simulink model "MMC_phase_centralized_HAAS_20260927"  (R2024b)
settings: Solver=FixedStepDiscrete  StartTime=t_init_sim  StopTime=sim_time  FixedStep=Ts  RelTol=1e-3
values from neighbouring files (symbols this model uses):
  a = 1    [script_MMC_phase_hackathon_NLM_centralized_HAAS_20260927.m]
  C1low1_active = 1    [script_MMC_phase_hackathon_NLM_centralized_HAAS_20260927.m]
  C2low1_active = 1    [script_MMC_phase_hackathon_NLM_centralized_HAAS_20260927.m]
  C_bus = 4400e-6    (= 0.0044)    [script_MMC_phase_hackathon_NLM_centralized_HAAS_20260927.m]
  C_M_extra = C_m-twist_high_side_C    [script_MMC_phase_hackathon_NLM_centralized_HAAS_20260927.m]
  duty_cycle = 1.0    (= 1)    [script_MMC_phase_hackathon_NLM_centralized_HAAS_20260927.m]
  f0 = 50    [script_MMC_phase_hackathon_NLM_centralized_HAAS_20260927.m]
  feeder_current_lower_rate_limit = -10    [script_MMC_phase_hackathon_NLM_centralized_HAAS_20260927.m]    (also in twist_parameters.m = -500)
  feeder_current_tab = [0.328 0.217 0.162 0.132 0.109 0.094 0.083 0.075 0.068 0.062 0.058 0.054 ... (42 elements, 14x3)]    [feeder_current.mat]
  feeder_current_upper_rate_limit = 0.386/(20e-3)    (= 19.3)    [twist_parameters.m]
  is6VExternallySupplied = true    [script_MMC_phase_hackathon_NLM_centralized_HAAS_20260927.m]
  isFeederJumperOpen = true    [script_MMC_phase_hackathon_NLM_centralized_HAAS_20260927.m]
  L_arm = 30e-3    (= 0.03)    [script_MMC_phase_hackathon_NLM_centralized_HAAS_20260927.m]
  m = 1    [script_MMC_phase_hackathon_NLM_centralized_HAAS_20260927.m]
  N = 5    [script_MMC_phase_hackathon_NLM_centralized_HAAS_20260927.m]
  power_losses = false    [script_MMC_phase_hackathon_NLM_centralized_HAAS_20260927.m]
  R = 15    [script_MMC_phase_hackathon_NLM_centralized_HAAS_20260927.m]
  R_arm = 0.2    [script_MMC_phase_hackathon_NLM_centralized_HAAS_20260927.m]
  source_V = 0    [script_MMC_phase_hackathon_NLM_centralized_HAAS_20260927.m]
  Tcom_sample = round(Tcom / Ts)    [script_MMC_phase_hackathon_NLM_centralized_HAAS_20260927.m]
  time_charge = 0.1    [script_MMC_phase_hackathon_NLM_centralized_HAAS_20260927.m]
  time_decharge = 1.5    [script_MMC_phase_hackathon_NLM_centralized_HAAS_20260927.m]
  Ts = 1e-6    (= 1e-06)    [script_MMC_phase_hackathon_NLM_centralized_HAAS_20260927.m]
  twist_data_acquisition_delay = 50e-9    (= 5e-08)    [script_MMC_phase_hackathon_NLM_centralized_HAAS_20260927.m]    (also in twist_parameters.m)
  twist_data_sampling_period = 1/twist_freq_data_sampling    (= 5e-05)    [script_MMC_phase_hackathon_NLM_centralized_HAAS_20260927.m]    (also in twist_parameters.m)
  twist_dead_time = 200e-9    (= 2e-07)    [twist_parameters.m]
  twist_freq_switching = 200e3    (= 200000)    [twist_parameters.m]
  twist_high_side_adc_R = 1/(1/2e6 + 1/2e6 + 1/(330e3+5.6e3))    (= 251272.836178)    [twist_parameters.m]
  twist_high_side_C = 33e-6*4 + 4.7e-6*12    (= 0.0001884)    [twist_parameters.m]
  twist_high_side_feeder_R = 47e3+4.7e3    (= 51700)    [twist_parameters.m]
  twist_high_side_rC = 0.1    [twist_parameters.m]
  twist_low_side_adc_R = 150e3+470    (= 150470)    [twist_parameters.m]
  twist_low_side_C_ceramic = 3*4.7e-6    (= 1.41e-05)    [twist_parameters.m]
  twist_low_side_C_electrolytic = 47e-6    (= 4.7e-05)    [twist_parameters.m]
  twist_low_side_L = 33e-6    (= 3.3e-05)    [twist_parameters.m]
  twist_low_side_rC = 700e-3    (= 0.7)    [twist_parameters.m]
  twist_low_side_rL = 20e-3    (= 0.02)    [twist_parameters.m]
  twist_R_VCC = (tau_VCC/twist_high_side_C  - twist_high_side_rC)/(1-(tau_VCC/twist_high_side_C - twist_high_side_rC)/R_parallel)    (= 1110.74997822)    [twist_parameters.m]
  VDC = 48    [script_MMC_phase_hackathon_NLM_centralized_HAAS_20260927.m]
undefined symbols (not defined in the file or in its folder): C_SM, feeder_current, gcbh, sps_rtmsupport, twist_low_side_lC
libraries: spsSeriesRLCBranchLib x135, spsTriangleGeneratorLib x60, spsMosfetLib x60, spsCurrentMeasurementLib x43, spsVoltageMeasurementLib x35, spsControlledCurrentSourceLib x30, spsDiodeLib x22, spsIdealSwitchLib x20, spsControlledVoltageSourceLib x1, spsGroundLib x1, spspowerguiLib x1
(part 22 of 22)

== matlab function MMC_phase_centralized_HAAS_20260927/ /Communication_subsystem/Upper_arm/M1_Comm/Snapshot ==
  data: rx_signal input uint64; local_frame_snapshot input; rx_variables output single; sync input; round_done input
function rx_variables = Snapshot_block(rx_signal, local_frame_snapshot, sync, round_done)
%#codegen
%
% Snapshot block SSAF.
%
% Comportement voulu :
%   - pendant le round, les trames reçues mettent à jour working_bank ;
%   - local_frame_snapshot met à jour la donnée locale ;
%   - au front montant de sync, published_snapshot = working_bank ;
%   - le contrôle lit published_snapshot pendant la période de contrôle.
%
% round_done est conservé dans l'interface pour debug, mais la publication
% du snapshot se fait sur le front montant de sync.

% =========================
% Paramètres
% =========================
VC_LSB = single(0.1);
I_LSB  = single(0.1);

% =========================
% Etats persistants
% =========================
persistent working_bank
persistent published_snapshot
persistent sync_z
persistent last_rx_word
persistent last_rx_valid

if isempty(working_bank)
    working_bank = zeros(12, 1, 'single');
end

if isempty(published_snapshot)
    published_snapshot = zeros(12, 1, 'single');
end

if isempty(sync_z)
    sync_z = false;
end

if isempty(last_rx_word)
    last_rx_word = uint64(0);
end

if isempty(last_rx_valid)
    last_rx_valid = false;
end

% =========================
% Détection fronts sync
% =========================
sync_bool = sync ~= 0;
rise_sync = sync_bool && ~sync_z;

% =========================================================
% 1) Publication du snapshot au front montant
%
% Important :
%   published_snapshot est mis à jour AVANT la sortie.
%   Il contient les données reçues jusqu'au pas précédent.
%   Une trame qui arrive exactement au même pas que rise_sync est traitée
%   plus bas et sera donc visible au prochain front montant.
% =========================================================
if rise_sync
    published_snapshot = working_bank;
end

% =========================================================
% 2) Sortie enregistrée
%
% rx_variables ne dépend pas directement de rx_signal ou
% local_frame_snapshot au même pas de simulation.
% Cela évite une boucle algébrique avec le CVB.
% =========================================================
rx_variables = published_snapshot;

% Petit usage de round_done pour éviter qu'il soit complètement inutilisé.
% Il ne déclenche pas la publication.
if round_done ~= 0
    published_snapshot = published_snapshot;
end

% =========================
% 3) Mise à jour avec la trame locale
%
% local_frame_snapshot est émis seulement quand un nouveau round démarre.
% =========================
local_word = uint64(local_frame_snapshot(1));

[local_valid, local_current_present, local_id, local_vc, local_iarm] = ...
    unpack_frame(local_word, VC_LSB, I_LSB);

if local_valid
    working_bank = update_bank_from_frame(working_bank, ...
                                          local_valid, ...
                                          local_current_present, ...
                                          local_id, ...
                                          local_vc, ...
                                          local_iarm);
end

% =========================
% 4) Mise à jour avec la trame reçue depuis l'anneau
% =========================
rx_word = uint64(rx_signal(1));

[rx_valid, rx_current_present, rx_id, rx_vc, rx_iarm] = ...
    unpack_frame(rx_word, VC_LSB, I_LSB);

new_rx = rx_valid && ((rx_word ~= last_rx_word) || ~last_rx_valid);

if new_rx
    working_bank = update_bank_from_frame(working_bank, ...
                                          rx_valid, ...
                                          rx_current_present, ...
                                          rx_id, ...
                                          rx_vc, ...
                                          rx_iarm);
end

% =========================
% Mise à jour mémoires
% =========================
sync_z = sync_bool;

last_rx_word  = rx_word;
last_rx_valid = rx_valid;


% =========================================================
% UPDATE BANK FROM FRAME
% =========================================================
function bank_out = update_bank_from_frame(bank_in, valid, current_present, id, vc, iarm)
%#codegen

    bank_out = bank_in;

    if ~valid
        return;
    end

    % Upper arm : ID 1 à 5
    if id >= uint8(1) && id <= uint8(5)

        idx = double(id);          % ID 1 -> bank(1), ..., ID 5 -> bank(5)
        bank_out(idx) = single(vc);

        % Seul M1 transporte I_u
        if id == uint8(1) && current_present
            bank_out(6) = single(iarm);
        end

    % Lower arm : ID 6 à 10
    elseif id >= uint8(6) && id <= uint8(10)

        idx = 6 + double(id - uint8(5));  % ID 6 -> bank(7), ..., ID 10 -> bank(11)
        bank_out(idx) = single(vc);

        % Seul M6 transporte I_l
        if id == uint8(6) && current_present
            bank_out(12) = single(iarm);
        end
    end
end


% =========================================================
% UNPACK FRAME
%
% Format uint64:
%   bit 41      : valid
%   bit 40      : current_present
%   bits 39..32 : node_id
%   bits 31..16 : Vc local, uint16
%   bits 15..0  : I arm, int16 encodé en complément à deux
% =========================================================
function [valid, current_present, id, vc, iarm] = unpack_frame(frame, vc_lsb, i_lsb)
%#codegen

    frame_scalar = uint64(frame(1));

    valid = bitand(bitshift(frame_scalar, -41), uint64(1)) ~= uint64(0);
    current_present = bitand(bitshift(frame_scalar, -40), uint64(1)) ~= uint64(0);

    id = uint8(bitand(bitshift(frame_scalar, -32), uint64(255)));

    vc_q = uint16(bitand(bitshift(frame_scalar, -16), uint64(65535)));
    vc = single(double(vc_q) * double(vc_lsb));

    i_u16 = uint16(bitand(frame_scalar, uint64(65535)));

    if i_u16 >= uint16(32768)
        i_q_double = double(i_u16) - 65536;
    else
        i_q_double = double(i_u16);
    end

    iarm = single(i_q_double * double(i_lsb));
end

end

== matlab function MMC_phase_centralized_HAAS_20260927/ /Subsystem/Subsystem1/Hardware M4/Power losses branch 1/Branch switching loss ==
  data: VHigh input; twist_FET_Psw output; ILow input
function twist_FET_Psw = powerLossesSwitch(VHigh, ILow)
    %Twist switch power losses
    twist_freq_switching = 200e3;
    twist_FET_trise = 17e-9;
    twist_FET_tfall = 9e-9;

    twist_FET_Psw = 1/2*VHigh*ILow*twist_freq_switching*(twist_FET_trise + twist_FET_tfall);
end

== matlab function MMC_phase_centralized_HAAS_20260927/ /Subsystem/Subsystem1/Hardware M4/Power losses branch 2/Branch DT loss ==
  data: twist_FET_Pdt output; ILow input
function twist_FET_Pdt = powerLossesDeadTime(ILow)
    %Twist gate power losses
    twist_freq_switching = 200e3;
    twist_FET_Vf = 1.2;
    twist_FET_tDr = 10e-9;
    twist_FET_tDf = 0;

    twist_FET_Pdt = twist_FET_Vf*ILow*(twist_FET_tDr+twist_FET_tDf)*twist_freq_switching;
end

== matlab function MMC_phase_centralized_HAAS_20260927/ /Subsystem/Subsystem/Hardware M2/Feeder block/MATLAB Function ==
  data: i_feeder input; vC input; isfeederdisabled input; active_1 input; y output; Q_VCC output
function [y,Q_VCC]  = feeder_characteristics(i_feeder,vC,isfeederdisabled,active_1)

if(isfeederdisabled == 1)
    if(vC>=9.7)
        y = 11.2e-3;
        Q_VCC = 0;
    elseif(vC>=8.9 && vC < 9.7)
        if(active_1 == true)
            y = 11.2e-3;
            Q_VCC = 0;
        else
            y = 0;
            Q_VCC = 1;
        end
    else
        y = 0;
        Q_VCC = 1;
    end
else
    if(vC>=9.7)
        y = i_feeder;
        Q_VCC = 0;
    elseif(vC>=8.9 && vC < 9.7)
        if(active_1 == true)
            y = i_feeder;
            Q_VCC = 0;
        else
            y = 0;
            Q_VCC = 1;
        end
    else
        y = 0;
        Q_VCC = 1;
    end
end

== matlab function MMC_phase_centralized_HAAS_20260927/ /Subsystem/Subsystem1/Hardware M4/Power losses branch 2/Branch cond loss ==
  data: twist_FET_Pcond output; VHigh input; VLow input; ILow input
function twist_FET_Pcond = powerLossesCond(VHigh, VLow, ILow)
    %Twist conduction power losses
    twist_FET_Ron = 0.025;

    twist_FET_PcondH = pow2(ILow)*twist_FET_Ron*(VLow/VHigh);
    twist_FET_PcondL = pow2(ILow)*twist_FET_Ron*(1 - VLow/VHigh);

    twist_FET_Pcond = twist_FET_PcondH + twist_FET_PcondL;
end

== matlab function MMC_phase_centralized_HAAS_20260927/ /Subsystem/Subsystem1/Hardware M4/Power losses branch 2/Branch gate loss ==
  data: twist_FET_Pg output
function twist_FET_Pg = powerLossesGate()
    %Twist gate power losses
    twist_freq_switching = 200e3;
    twist_FET_QgH = 31e-9;
    twist_FET_QgL = 31e-9;
    twist_FET_Vgs = 11;

    twist_FET_Pg = (twist_FET_QgH + twist_FET_QgL)*twist_FET_Vgs*twist_freq_switching;
end

== matlab function MMC_phase_centralized_HAAS_20260927/ /Subsystem/Subsystem1/Hardware M4/Power losses branch 2/Branch switching loss ==
  data: VHigh input; twist_FET_Psw output; ILow input
function twist_FET_Psw = powerLossesSwitch(VHigh, ILow)
    %Twist switch power losses
    twist_freq_switching = 200e3;
    twist_FET_trise = 17e-9;
    twist_FET_tfall = 9e-9;

    twist_FET_Psw = 1/2*VHigh*ILow*twist_freq_switching*(twist_FET_trise + twist_FET_tfall);
end

== matlab function MMC_phase_centralized_HAAS_20260927/ /Subsystem/Subsystem1/Hardware M5/Feeder block/MATLAB Function ==
  data: i_feeder input; vC input; isfeederdisabled input; active_1 input; y output; Q_VCC output
function [y,Q_VCC]  = feeder_characteristics(i_feeder,vC,isfeederdisabled,active_1)

if(isfeederdisabled == 1)
    if(vC>=9.7)
        y = 11.2e-3;
        Q_VCC = 0;
    elseif(vC>=8.9 && vC < 9.7)
        if(active_1 == true)
            y = 11.2e-3;
            Q_VCC = 0;
        else
            y = 0;
            Q_VCC = 1;
        end
    else
        y = 0;
        Q_VCC = 1;
    end
else
    if(vC>=9.7)
        y = i_feeder;
        Q_VCC = 0;
    elseif(vC>=8.9 && vC < 9.7)
        if(active_1 == true)
            y = i_feeder;
            Q_VCC = 0;
        else
            y = 0;
            Q_VCC = 1;
        end
    else
        y = 0;
        Q_VCC = 1;
    end
end

== matlab function MMC_phase_centralized_HAAS_20260927/ /Subsystem/Subsystem1/Hardware M5/Power losses branch 1/Branch DT loss ==
  data: twist_FET_Pdt output; ILow input
function twist_FET_Pdt = powerLossesDeadTime(ILow)
    %Twist gate power losses
    twist_freq_switching = 200e3;
    twist_FET_Vf = 1.2;
    twist_FET_tDr = 10e-9;
    twist_FET_tDf = 0;

    twist_FET_Pdt = twist_FET_Vf*ILow*(twist_FET_tDr+twist_FET_tDf)*twist_freq_switching;
end

== matlab function MMC_phase_centralized_HAAS_20260927/ /Subsystem/Subsystem1/Hardware M5/Power losses branch 1/Branch cond loss ==
  data: twist_FET_Pcond output; VHigh input; VLow input; ILow input
function twist_FET_Pcond = powerLossesCond(VHigh, VLow, ILow)
    %Twist conduction power losses
    twist_FET_Ron = 0.025;

    twist_FET_PcondH = pow2(ILow)*twist_FET_Ron*(VLow/VHigh);
    twist_FET_PcondL = pow2(ILow)*twist_FET_Ron*(1 - VLow/VHigh);

    twist_FET_Pcond = twist_FET_PcondH + twist_FET_PcondL;
end

== matlab function MMC_phase_centralized_HAAS_20260927/ /Subsystem/Subsystem1/Hardware M5/Power losses branch 1/Branch gate loss ==
  data: twist_FET_Pg output
function twist_FET_Pg = powerLossesGate()
    %Twist gate power losses
    twist_freq_switching = 200e3;
    twist_FET_QgH = 31e-9;
    twist_FET_QgL = 31e-9;
    twist_FET_Vgs = 11;

    twist_FET_Pg = (twist_FET_QgH + twist_FET_QgL)*twist_FET_Vgs*twist_freq_switching;
end

== matlab function MMC_phase_centralized_HAAS_20260927/ /Subsystem/Subsystem1/Hardware M5/Power losses branch 1/Branch switching loss ==
  data: VHigh input; twist_FET_Psw output; ILow input
function twist_FET_Psw = powerLossesSwitch(VHigh, ILow)
    %Twist switch power losses
    twist_freq_switching = 200e3;
    twist_FET_trise = 17e-9;
    twist_FET_tfall = 9e-9;

    twist_FET_Psw = 1/2*VHigh*ILow*twist_freq_switching*(twist_FET_trise + twist_FET_tfall);
end

== matlab function MMC_phase_centralized_HAAS_20260927/ /Subsystem/Subsystem1/Hardware M5/Power losses branch 2/Branch DT loss ==
  data: twist_FET_Pdt output; ILow input
function twist_FET_Pdt = powerLossesDeadTime(ILow)
    %Twist gate power losses
    twist_freq_switching = 200e3;
    twist_FET_Vf = 1.2;
    twist_FET_tDr = 10e-9;
    twist_FET_tDf = 0;

    twist_FET_Pdt = twist_FET_Vf*ILow*(twist_FET_tDr+twist_FET_tDf)*twist_freq_switching;
end

== matlab function MMC_phase_centralized_HAAS_20260927/ /Subsystem/Subsystem1/Hardware M5/Power losses branch 2/Branch cond loss ==
  data: twist_FET_Pcond output; VHigh input; VLow input; ILow input
function twist_FET_Pcond = powerLossesCond(VHigh, VLow, ILow)
    %Twist conduction power losses
    twist_FET_Ron = 0.025;

    twist_FET_PcondH = pow2(ILow)*twist_FET_Ron*(VLow/VHigh);
    twist_FET_PcondL = pow2(ILow)*twist_FET_Ron*(1 - VLow/VHigh);

    twist_FET_Pcond = twist_FET_PcondH + twist_FET_PcondL;
end

== matlab function MMC_phase_centralized_HAAS_20260927/ /Subsystem/Subsystem1/Hardware M5/Power losses branch 2/Branch gate loss ==
  data: twist_FET_Pg output
function twist_FET_Pg = powerLossesGate()
    %Twist gate power losses
    twist_freq_switching = 200e3;
    twist_FET_QgH = 31e-9;
    twist_FET_QgL = 31e-9;
    twist_FET_Vgs = 11;

    twist_FET_Pg = (twist_FET_QgH + twist_FET_QgL)*twist_FET_Vgs*twist_freq_switching;
end

== matlab function MMC_phase_centralized_HAAS_20260927/ /Subsystem/Subsystem1/Hardware M5/Power losses branch 2/Branch switching loss ==
  data: VHigh input; twist_FET_Psw output; ILow input
function twist_FET_Psw = powerLossesSwitch(VHigh, ILow)
    %Twist switch power losses
    twist_freq_switching = 200e3;
    twist_FET_trise = 17e-9;
    twist_FET_tfall = 9e-9;

    twist_FET_Psw = 1/2*VHigh*ILow*twist_freq_switching*(twist_FET_trise + twist_FET_tfall);
end

== matlab function MMC_phase_centralized_HAAS_20260927/ /Sinus Modulation + Sorting Algorithm/M2 MCU/CVB_upper ==
  data: g input; y output; M_number input
function y = fcn(g,M_number)

Gp = zeros(1,2);

Gp(1)=g(2*M_number-1);
Gp(2)=g(2*M_number);

y=Gp';
